simulink model "Ejercicio_5_4"  (R2026b)
settings: Solver=VariableStepAuto  StopTime=t_stop
InitFcn:
  | caso_run = '5.4'; pv_params; clear caso_run
values from neighbouring files (symbols this model uses):
  alpha0 = fzero(f, [0 1])    [pv_params(1).m]    (also in pv_params(2).m; pv_params(3).m; pv_params(4).m; pv_params.m)
  comedelay = 20e-3    (= 0.02)    [pv_params(1).m]    (also in pv_params(2).m; pv_params(3).m; pv_params(4).m; pv_params.m)
  dSOC = 0.01    [pv_params(1).m]    (also in pv_params(2).m; pv_params(3).m; pv_params(4).m; pv_params.m)
  E_bat = 1000    [pv_params(1).m]    (also in pv_params(2).m; pv_params(3).m; pv_params(4).m; pv_params.m)
  eta_bat = 0.95    [pv_params(1).m]    (also in pv_params(2).m; pv_params(3).m; pv_params(4).m; pv_params.m)
  Pbat_max = 3000    [pv_params(1).m]    (also in pv_params(2).m; pv_params(3).m; pv_params(4).m; pv_params.m)
  Pinv_nom = 2000    [pv_params(1).m]    (also in pv_params(2).m; pv_params(3).m; pv_params(4).m; pv_params.m)
  Ppcc0 = sum(min(alpha0*Pinv_nom, Pavail))    [pv_params(1).m]    (also in pv_params(2).m; pv_params(3).m; pv_params(4).m; pv_params.m)
  SOC0 = 0.8    [pv_params(1).m]    (also in pv_params(2).m; pv_params(3).m; pv_params(4).m; pv_params.m)
  SOCmax = 0.9    [pv_params(1).m]    (also in pv_params(2).m; pv_params(3).m; pv_params(4).m; pv_params.m)
  SOCmin = 0.1    [pv_params(1).m]    (also in pv_params(2).m; pv_params(3).m; pv_params(4).m; pv_params.m)
  t_sample_ppc = 0.2    [pv_params(1).m]    (also in pv_params(2).m; pv_params(3).m; pv_params(4).m; pv_params.m)
  tau_bat = 0.2    [pv_params(1).m]    (also in pv_params(2).m; pv_params(3).m; pv_params(4).m; pv_params.m)
  tau_pv = 0.5    [pv_params(1).m]    (also in pv_params(2).m; pv_params(3).m; pv_params(4).m; pv_params.m)
libraries: sl_discontinuities x6
settings Model: Creator=mithu  LastModifiedBy=mithu

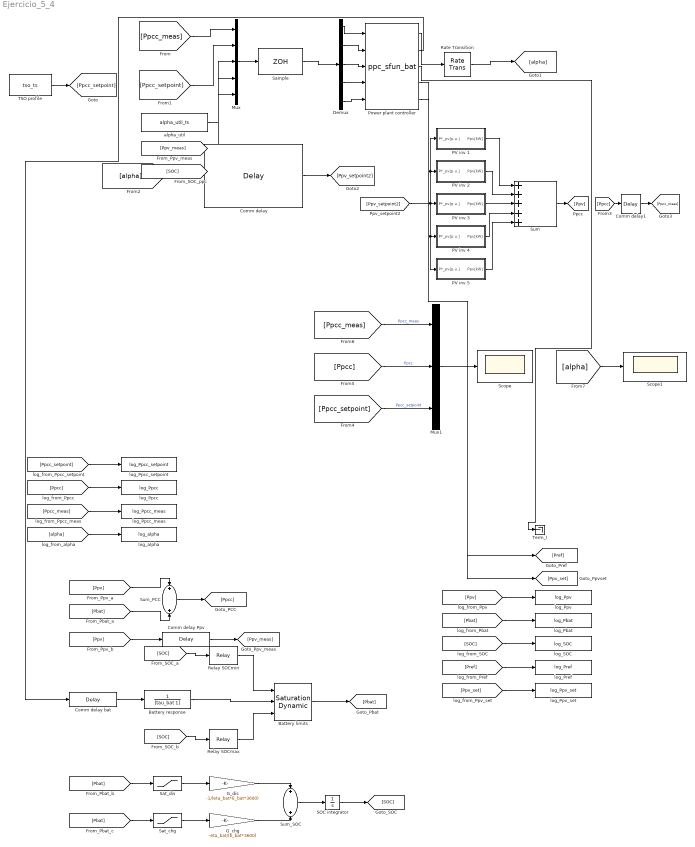
== system Ejercicio_5_4 ==
  Battery limits : sl_discontinuities/Saturation Dynamic  OutMin=[]  OutMax=[]  OutDataTypeStr=Inherit: Same as second input  OutDataType=fixdt(1, 16)  OutScaling=2^-10  DoSatur=off
      settings: LibrarySourceBlock=|
      | simulink/Discontinuities/Saturation
      | Dynamic
  Battery response : TransferFcn  Numerator=1  Denominator=[tau_bat 1]
  Comm delay : TransportDelay  DelayTime=comedelay  InitialOutput=alpha0
  Comm delay Ppv : TransportDelay  DelayTime=comedelay  InitialOutput=Ppcc0
  Comm delay bat : TransportDelay  DelayTime=comedelay
  Comm delay1 : TransportDelay  DelayTime=comedelay  InitialOutput=Ppcc0
  Demux : Demux  Outputs=5
  G_chg : Gain  Gain=-eta_bat/(E_bat*3600)
  G_dis : Gain  Gain=-1/(eta_bat*E_bat*3600)
  Mux : Mux  Inputs=5
  Mux1 : Mux  Inputs=3
  PV inv 1 : Subsystem
  PV inv 2 : Subsystem
  PV inv 3 : Subsystem
  PV inv 4 : Subsystem
  PV inv 5 : Subsystem
  Power plant controller : M-S-Function  FunctionName=ppc_sfun_bat  Parameters=t_sample_ppc, Kp, Ki, Ppv_nom, ctrl5, I0, Pref0, ramp_kWmin, Pbat_max, SOCmin, SOCmax
  Rate Transition : RateTransition  Integrity=off  InitialCondition=alpha0
  Relay SOCmax : Relay  OnSwitchValue=SOCmax  OffSwitchValue=SOCmax-dSOC  OnOutputValue=0  OffOutputValue=-Pbat_max
  Relay SOCmin : Relay  OnSwitchValue=SOCmin+dSOC  OffSwitchValue=SOCmin  OnOutputValue=Pbat_max
  SOC integrator : Integrator  InitialCondition=SOC0
  Sample : ZeroOrderHold  SampleTime=t_sample_ppc
  Sat_chg : Saturate  UpperLimit=0  LowerLimit=-1e9
  Sat_dis : Saturate  UpperLimit=1e9  LowerLimit=0
  Scope : Scope
      settings: ActiveDisplayYMinimum=4375  ActiveDisplayYMaximum=10625.000000000004
  Scope1 : Scope
      settings: ActiveDisplayYMinimum=0.4375  ActiveDisplayYMaximum=1.0625
  Sum : Sum  Inputs=+++++
  Sum_PCC : Sum
  Sum_SOC : Sum
  TSO profile : FromWorkspace  VariableName=tso_ts  Interpolate=off  OutputAfterFinalValue=Holding final value
  Term_I : Terminator
  alpha_util : FromWorkspace  VariableName=alpha_util_ts  OutputAfterFinalValue=Holding final value
  log_Pbat : ToWorkspace  VariableName=log_Pbat  SaveFormat=Timeseries  SampleTime=-1
  log_Ppcc : ToWorkspace  VariableName=log_Ppcc  SaveFormat=Timeseries  SampleTime=-1
  log_Ppcc_meas : ToWorkspace  VariableName=log_Ppcc_meas  SaveFormat=Timeseries  SampleTime=-1
  log_Ppcc_setpoint : ToWorkspace  VariableName=log_Ppcc_setpoint  SaveFormat=Timeseries  SampleTime=-1
  log_Ppv : ToWorkspace  VariableName=log_Ppv  SaveFormat=Timeseries  SampleTime=-1
  log_Ppv_set : ToWorkspace  VariableName=log_Ppv_set  SaveFormat=Timeseries  SampleTime=-1
  log_Pref : ToWorkspace  VariableName=log_Pref  SaveFormat=Timeseries  SampleTime=-1
  log_SOC : ToWorkspace  VariableName=log_SOC  SaveFormat=Timeseries  SampleTime=-1
  log_alpha : ToWorkspace  VariableName=log_alpha  SaveFormat=Timeseries  SampleTime=-1
  wires:
  [Ppcc_meas] -> Mux/1
  [Ppcc_setpoint] -> Mux/2
  Mux/1 -> Sample/1
  Sample/1 -> Demux/1
  Demux/1 -> Power plant controller/1
  Demux/2 -> Power plant controller/2
  Power plant controller/1 -> Rate Transition/1
  Rate Transition/1 -> [alpha]
  [alpha] -> Comm delay/1
  Comm delay/1 -> [Ppv_setpoint2]
  [Ppv_setpoint2] -> PV inv 1/1(P*_pv[p.u.]), PV inv 2/1(P*_pv[p.u.]), PV inv 5/1(P*_pv[p.u.]), PV inv 4/1(P*_pv[p.u.]), PV inv 3/1(P*_pv[p.u.])
  PV inv 1/1(Ppv[kW]) -> Sum/1
  PV inv 3/1(Ppv[kW]) -> Sum/3
  PV inv 4/1(Ppv[kW]) -> Sum/4
  PV inv 5/1(Ppv[kW]) -> Sum/5
  PV inv 2/1(Ppv[kW]) -> Sum/2
  Sum/1 -> [Ppv]
  [Ppcc] -> Comm delay1/1
  Comm delay1/1 -> [Ppcc_meas]
  [Ppcc_meas] -> Mux1/1  "Ppcc_meas"
  [Ppcc] -> Mux1/2  "Ppcc"
  [Ppcc_setpoint] -> Mux1/3  "Ppcc_setpoint"
  Mux1/1 -> Scope/1
  [alpha] -> Scope1/1
  [Ppcc_setpoint] -> log_Ppcc_setpoint/1
  [Ppcc] -> log_Ppcc/1
  [Ppcc_meas] -> log_Ppcc_meas/1
  [alpha] -> log_alpha/1
  TSO profile/1 -> [Ppcc_setpoint]
  alpha_util/1 -> Mux/3
  Demux/3 -> Power plant controller/3
  [Ppv_meas] -> Mux/4
  [SOC] -> Mux/5
  Demux/4 -> Power plant controller/4
  Demux/5 -> Power plant controller/5
  [Ppv] -> Sum_PCC/1
  [Pbat] -> Sum_PCC/2
  Sum_PCC/1 -> [Ppcc]
  [Ppv] -> Comm delay Ppv/1
  Comm delay Ppv/1 -> [Ppv_meas]
  Power plant controller/2 -> Comm delay bat/1
  Comm delay bat/1 -> Battery response/1
  Battery response/1 -> Battery limits/2
  [SOC] -> Relay SOCmin/1
  Relay SOCmin/1 -> Battery limits/1
  [SOC] -> Relay SOCmax/1
  Relay SOCmax/1 -> Battery limits/3
  Battery limits/1 -> [Pbat]
  [Pbat] -> Sat_dis/1
  Sat_dis/1 -> G_dis/1
  G_dis/1 -> Sum_SOC/1
  [Pbat] -> Sat_chg/1
  Sat_chg/1 -> G_chg/1
  G_chg/1 -> Sum_SOC/2
  Sum_SOC/1 -> SOC integrator/1
  SOC integrator/1 -> [SOC]
  Power plant controller/3 -> Term_I/1
  Power plant controller/4 -> [Pref]
  Power plant controller/5 -> [Ppv_set]
  [Ppv] -> log_Ppv/1
  [Pbat] -> log_Pbat/1
  [SOC] -> log_SOC/1
  [Pref] -> log_Pref/1
  [Ppv_set] -> log_Ppv_set/1

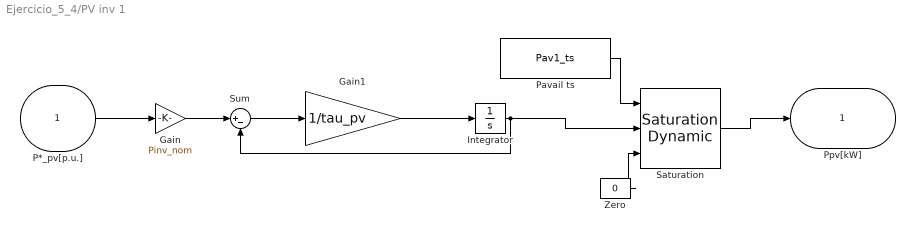
== system Ejercicio_5_4/PV inv 1 ==
  P*_pv[p.u.] : Inport
  Gain : Gain  Gain=Pinv_nom
  Gain1 : Gain  Gain=1/tau_pv
  Integrator : Integrator  InitialCondition=alpha0*Pinv_nom
  Pavail ts : FromWorkspace  VariableName=Pav1_ts  OutputAfterFinalValue=Holding final value
  Saturation : sl_discontinuities/Saturation Dynamic  OutMin=[]  OutMax=[]  OutDataTypeStr=Inherit: Same as second input  OutDataType=fixdt(1, 16)  OutScaling=2^-10  DoSatur=off
      settings: LibrarySourceBlock=|
      | simulink/Discontinuities/Saturation
      | Dynamic
  Sum : Sum  Inputs=|+-
  Zero : Constant  Value=0
  Ppv[kW] : Outport
  wires:
  P*_pv[p.u.]/1 -> Gain/1
  Gain/1 -> Sum/1
  Sum/1 -> Gain1/1
  Gain1/1 -> Integrator/1
  Integrator/1 -> Saturation/2, Sum/2
  Pavail ts/1 -> Saturation/1
  Zero/1 -> Saturation/3
  Saturation/1 -> Ppv[kW]/1

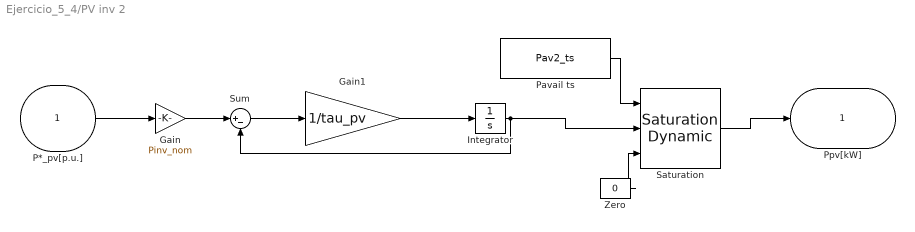
== system Ejercicio_5_4/PV inv 2 ==
  P*_pv[p.u.] : Inport
  Gain : Gain  Gain=Pinv_nom
  Gain1 : Gain  Gain=1/tau_pv
  Integrator : Integrator  InitialCondition=alpha0*Pinv_nom
  Pavail ts : FromWorkspace  VariableName=Pav2_ts  OutputAfterFinalValue=Holding final value
  Saturation : sl_discontinuities/Saturation Dynamic  OutMin=[]  OutMax=[]  OutDataTypeStr=Inherit: Same as second input  OutDataType=fixdt(1, 16)  OutScaling=2^-10  DoSatur=off
      settings: LibrarySourceBlock=|
      | simulink/Discontinuities/Saturation
      | Dynamic
  Sum : Sum  Inputs=|+-
  Zero : Constant  Value=0
  Ppv[kW] : Outport
  wires:
  P*_pv[p.u.]/1 -> Gain/1
  Gain/1 -> Sum/1
  Sum/1 -> Gain1/1
  Gain1/1 -> Integrator/1
  Integrator/1 -> Saturation/2, Sum/2
  Pavail ts/1 -> Saturation/1
  Zero/1 -> Saturation/3
  Saturation/1 -> Ppv[kW]/1

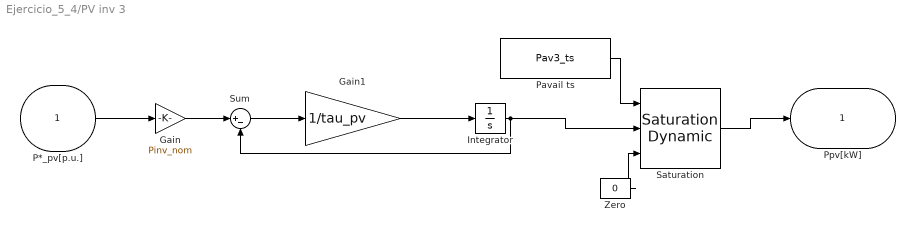
== system Ejercicio_5_4/PV inv 3 ==
  P*_pv[p.u.] : Inport
  Gain : Gain  Gain=Pinv_nom
  Gain1 : Gain  Gain=1/tau_pv
  Integrator : Integrator  InitialCondition=alpha0*Pinv_nom
  Pavail ts : FromWorkspace  VariableName=Pav3_ts  OutputAfterFinalValue=Holding final value
  Saturation : sl_discontinuities/Saturation Dynamic  OutMin=[]  OutMax=[]  OutDataTypeStr=Inherit: Same as second input  OutDataType=fixdt(1, 16)  OutScaling=2^-10  DoSatur=off
      settings: LibrarySourceBlock=|
      | simulink/Discontinuities/Saturation
      | Dynamic
  Sum : Sum  Inputs=|+-
  Zero : Constant  Value=0
  Ppv[kW] : Outport
  wires:
  P*_pv[p.u.]/1 -> Gain/1
  Gain/1 -> Sum/1
  Sum/1 -> Gain1/1
  Gain1/1 -> Integrator/1
  Integrator/1 -> Saturation/2, Sum/2
  Pavail ts/1 -> Saturation/1
  Zero/1 -> Saturation/3
  Saturation/1 -> Ppv[kW]/1

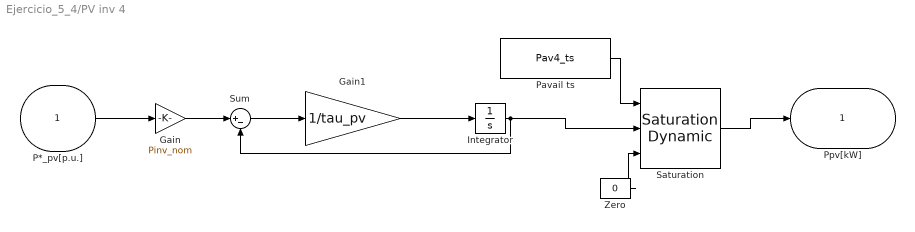
== system Ejercicio_5_4/PV inv 4 ==
  P*_pv[p.u.] : Inport
  Gain : Gain  Gain=Pinv_nom
  Gain1 : Gain  Gain=1/tau_pv
  Integrator : Integrator  InitialCondition=alpha0*Pinv_nom
  Pavail ts : FromWorkspace  VariableName=Pav4_ts  OutputAfterFinalValue=Holding final value
  Saturation : sl_discontinuities/Saturation Dynamic  OutMin=[]  OutMax=[]  OutDataTypeStr=Inherit: Same as second input  OutDataType=fixdt(1, 16)  OutScaling=2^-10  DoSatur=off
      settings: LibrarySourceBlock=|
      | simulink/Discontinuities/Saturation
      | Dynamic
  Sum : Sum  Inputs=|+-
  Zero : Constant  Value=0
  Ppv[kW] : Outport
  wires:
  P*_pv[p.u.]/1 -> Gain/1
  Gain/1 -> Sum/1
  Sum/1 -> Gain1/1
  Gain1/1 -> Integrator/1
  Integrator/1 -> Saturation/2, Sum/2
  Pavail ts/1 -> Saturation/1
  Zero/1 -> Saturation/3
  Saturation/1 -> Ppv[kW]/1

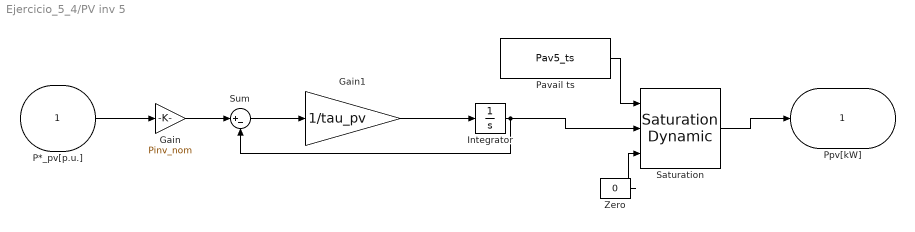
== system Ejercicio_5_4/PV inv 5 ==
  P*_pv[p.u.] : Inport
  Gain : Gain  Gain=Pinv_nom
  Gain1 : Gain  Gain=1/tau_pv
  Integrator : Integrator  InitialCondition=alpha0*Pinv_nom
  Pavail ts : FromWorkspace  VariableName=Pav5_ts  OutputAfterFinalValue=Holding final value
  Saturation : sl_discontinuities/Saturation Dynamic  OutMin=[]  OutMax=[]  OutDataTypeStr=Inherit: Same as second input  OutDataType=fixdt(1, 16)  OutScaling=2^-10  DoSatur=off
      settings: LibrarySourceBlock=|
      | simulink/Discontinuities/Saturation
      | Dynamic
  Sum : Sum  Inputs=|+-
  Zero : Constant  Value=0
  Ppv[kW] : Outport
  wires:
  P*_pv[p.u.]/1 -> Gain/1
  Gain/1 -> Sum/1
  Sum/1 -> Gain1/1
  Gain1/1 -> Integrator/1
  Integrator/1 -> Saturation/2, Sum/2
  Pavail ts/1 -> Saturation/1
  Zero/1 -> Saturation/3
  Saturation/1 -> Ppv[kW]/1
